simulink model "inverter_s1_kal"  (R2023b)
(part 2 of 3)

  N-Channel IGBT5 : ee_lib/Semiconductors & Converters/N-Channel IGBT  Commented=on  model_type=ee.enum.igbt.parameterization.equation  Ices=2 mA  Vces=600 V  Vth=6 V  Vce_sat=2.6 V  Ice_sat=400 A  Vge_sat=10 V  Tmeas=25 degC  Vge_vec=[-1, 0, 2, 3, 5, 6, 7, 8, 10, 12, 15, 18, 20] V  Vce_vec=[0, .25, .5, .75, 1, 1.26, 1.51, 1.76, 2.01, 2.26, 2.51, 2.76, 3.01, 3.27, 3.52, 3.77, 4.02, 4.27, 4.52, 4.77] V  T_vec=[25, 125] degC  Ic_mat=[0, 0, 0, 0, 0, 0, 0, 0, 0, 0, 0, 0, 0, 0, 0, 0, 0, 0, 0, 0; 0, 0, 0, 0, 0, 0, 0, 0, 0, 0, 0, 0, 0, 0, 0, 0, 0, 0, 0, 0; 0, 0, 0, 0, 0, 0, 0, 0, 0, 0, 0, 0, 0, 0, 0, 0, 0, 0, 0, 0; 0, 0, 0, 0, 0, 0, 0, 0, 0, 0, 0, 0, 0, 0, 0, 0, 0, 0, 0, 0; 0, 0, 0, 0, 0, 0, 0, 0, 0, 0, 0, 0, 0, 0, 0, 0, 0, 0, 0, 0; 0, 0, 0, .81, 3.13, 4.97, 6.03, 6.53, 6.84, 7.01, 7.19, 7.32, 7.44, 7.55, 7.67, 7.78, 7.89, 8, 8.07, 8.07; 0, 0, 0, 1.07, 5.5, 12.93, 22.09, 29.14, 35.27, 38.97, 41.37, 43.08, 44.52, 45.45, 46.28, 46.85, 47.41, 47.76, 48.06, 48.36; 0, 0, 0, 1.1, 6.99, 16.51, 28.38, 41.53, 55.76, 69.08, 80.5, 89.56, 96.13, 101.45, 105.15, 107.99, 110.09, 111.87, 113.54, 114.95; 0, 0, 0, 1.36, 6.26, 17.43, 33.6, 50.43, 71.75, 93.61, 114.64, 134.42, 151.44, 164.25, 177.06, 189.88, 202.69, 215.51, 228.32, 241.14; 0, 0, 0, 1.42, 6.4, 18.7, 36.19, 55.23, 79.71, 106.22, 131.28, 156.62, 182.79, 208.97, 235.15, 261.32, 287.5, 313.67, 339.85, 366.02; 0, 0, 0, 1.45, 6.81, 20.01, 39.61, 60.63, 88.74, 117.7, 147.16, 191.87, 237.14, 282.42, 327.69, 372.96, 418.23, 463.5, 508.77, 554.04; 0, 0, 0, 1.49, 6.97, 20.55, 41.34, 64.15, 94.91, 126.1, 170.16, 233.77, 297.38, 360.98, 424.59, 488.19, 551.8, 615.4, 679.01, 742.62; 0, 0, 0, 1.5, 7.5, 20.96, 42.17, 66.19, 98.34, 131.14, 187.84, 263.46, 339.09, 414.72, 490.34, 565.97, 641.6, 717.22, 792.85, 868.48] A  Ic_mat_3D=zeros(13, 20, 2) A  C_param=ee.enum.igbt.capacitanceParam.fixedciss  C_GE=23.7 nF  C_GC=2.7 nF  C_CE=0 nF  C_ies=26.4 nF  C_res=2.7 nF  C_oes=0 nF  C_GE_vec=[25, 31, 26.5, 24.9, 25, 24.9, 24.6, 24.7, 24.8] nF  C_GC_vec=[55, 9, 5.5, 3.1, 2.5, 2.1, 1.9, 1.8, 1.7] nF  C_Vge_vec=0 V  C_CE_vec=[5, 11, 6.5, 4.9, 3.5, 2.7, 2.1, 1.7, 1.4] nF  C_ies_vec=[80, 40, 32, 28, 27.5, 27, 26.5, 26.5, 26.5] nF  C_res_vec=[55, 9, 5.5, 3.1, 2.5, 2.1, 1.9, 1.8, 1.7] nF  C_oes_vec=[60, 20, 12, 8, 6, 4.8, 4, 3.5, 3.1] nF  C_Vce_vec=[0, 1, 2, 5, 10, 15, 20, 25, 30] V  charge_linearity_param=ee.enum.igbt.cgcLinearity.constant  C_OX=20 nF  V_C_OX=-5 V  TF=0 us  TT=0 us  ec=1  VAF=200 V  RC=0.001 Ohm  RE=0.001 Ohm  RG=0.001 Ohm  BF=50  T_param=ee.enum.igbt.temperatureParameterization.none  Ices_T2=100 mA  EG=1.11 eV  Vce_sat_T2=3 V  Tmeas2=125 degC  XTI=3  BEX=-1.5  RG_alpha=0 1/K  Tdevice=Tj_operating_K K  Tdevice_3D=25 degC  has_thermal_port=1  ig_specify=off  ig_priority=None  ig=0 A  ig_nominal_specify=off  ig_nominal_unit=A  ig_nominal_value=1  ic_specify=off  ic_priority=None  ic=0 A  ic_nominal_specify=off  ic_nominal_unit=A  ic_nominal_value=1  vge_specify=off  vge_priority=None  vge=0 V  vge_nominal_specify=off  vge_nominal_unit=V  vge_nominal_value=1  vce_specify=off  vce_priority=None  vce=0 V  vce_nominal_specify=off  vce_nominal_unit=V  vce_nominal_value=1  v_Cge_specify=off  v_Cge_priority=High  v_Cge=0 V  v_Cge_nominal_specify=off  v_Cge_nominal_unit=V  v_Cge_nominal_value=1  v_Cce_specify=off  v_Cce_priority=High  v_Cce=0 V  v_Cce_nominal_specify=off  v_Cce_nominal_unit=V  v_Cce_nominal_value=1  thermal_network_parameterization=ee.enum.thermalNetworkTopology.junctionCase  Rth=[0, 10] K/W  Rth_Cauer=[1, 3, 10] K/W  Rth_Foster=[4, 6] K/W  thermal_mass_parameterization=ee.enum.thermalNetwork.timeconstant  thermal_mass=[0, 1] J/K  thermal_mass_Cauer=[.1, .3, 1] J/K  thermal_mass_Foster=[1.5, 3] J/K  thermal_time_constant=[0, 10] s  thermal_time_constant_Cauer=[1, 3, 10] s  thermal_time_constant_Foster=[6, 18] s  thermal_mass_initial_temperatures=[25, 25] degC  thermal_mass_initial_temperatures_Cauer=[25, 25, 25] degC  Tvec_initial_Foster=[25, 25, 25, 25] degC  Ic_vec1=S12_Ic_cond A  Vce_vec1=[0, 1.1, 1.3, 1.45, 1.75, 2.25, 2.7] V  Rmiller=S12_Rmiller Ohm  Goff=S12_Goff 1/Ohm  t_on=S12_tondly s  t_rise=S12_risetime s  t_off=S12_toffdly s  t_fall=S12_falltime s  v_meas=S12_Voff_ref V  vStartTurnOn_specify=off  vStartTurnOn_priority=None  vStartTurnOn=1 V  tStartTurnOn_specify=off  tStartTurnOn_priority=None  tStartTurnOn=0 s  vStartTurnOff_specify=off  vStartTurnOff_priority=None  vStartTurnOff=0.5 V  tStartTurnOff_specify=off  tStartTurnOff_priority=None  tStartTurnOff=0 s  Tj_vec1=S12_Tj_cond K  Vce_mat1=S12_Vce_cond V  Tj_vec_loss=S12_Tj_loss K  Ic_vec_loss=S12_Ic_loss A  E_turn_on_mat1=S12_Eon J  E_turn_off_mat1=S12_Eoff J  iStartTurnOff_specify=off  iStartTurnOff_priority=None  iStartTurnOff=0 A  Tdevice_specify=off  Tdevice_priority=None
      settings: InternalSimscapePortConfiguration="{\"Bottom\":[],\"Left\":[{\"id\":\"G\",\"label\":\"\",\"type\":\"foundation.electrical.electrical\"},{\"id\":\"H\",\"label\":\"\",\"type\":\"foundation.thermal.thermal\"}],\"Right\":[{\"id\":\"C\",\"label\":\"\",\"type\":\"foundation.electrical.electrical\"},{\"id\":\"E\",\"label\":\"\",\"type\":\"foundation.electrical.electrical\"}],\"Top\":[]}"
  N-Channel IGBT6 : ee_lib/Semiconductors & Converters/N-Channel IGBT  Commented=on  model_type=ee.enum.igbt.parameterization.equation  Ices=2 mA  Vces=600 V  Vth=6 V  Vce_sat=2.6 V  Ice_sat=400 A  Vge_sat=10 V  Tmeas=25 degC  Vge_vec=[-1, 0, 2, 3, 5, 6, 7, 8, 10, 12, 15, 18, 20] V  Vce_vec=[0, .25, .5, .75, 1, 1.26, 1.51, 1.76, 2.01, 2.26, 2.51, 2.76, 3.01, 3.27, 3.52, 3.77, 4.02, 4.27, 4.52, 4.77] V  T_vec=[25, 125] degC  Ic_mat=[0, 0, 0, 0, 0, 0, 0, 0, 0, 0, 0, 0, 0, 0, 0, 0, 0, 0, 0, 0; 0, 0, 0, 0, 0, 0, 0, 0, 0, 0, 0, 0, 0, 0, 0, 0, 0, 0, 0, 0; 0, 0, 0, 0, 0, 0, 0, 0, 0, 0, 0, 0, 0, 0, 0, 0, 0, 0, 0, 0; 0, 0, 0, 0, 0, 0, 0, 0, 0, 0, 0, 0, 0, 0, 0, 0, 0, 0, 0, 0; 0, 0, 0, 0, 0, 0, 0, 0, 0, 0, 0, 0, 0, 0, 0, 0, 0, 0, 0, 0; 0, 0, 0, .81, 3.13, 4.97, 6.03, 6.53, 6.84, 7.01, 7.19, 7.32, 7.44, 7.55, 7.67, 7.78, 7.89, 8, 8.07, 8.07; 0, 0, 0, 1.07, 5.5, 12.93, 22.09, 29.14, 35.27, 38.97, 41.37, 43.08, 44.52, 45.45, 46.28, 46.85, 47.41, 47.76, 48.06, 48.36; 0, 0, 0, 1.1, 6.99, 16.51, 28.38, 41.53, 55.76, 69.08, 80.5, 89.56, 96.13, 101.45, 105.15, 107.99, 110.09, 111.87, 113.54, 114.95; 0, 0, 0, 1.36, 6.26, 17.43, 33.6, 50.43, 71.75, 93.61, 114.64, 134.42, 151.44, 164.25, 177.06, 189.88, 202.69, 215.51, 228.32, 241.14; 0, 0, 0, 1.42, 6.4, 18.7, 36.19, 55.23, 79.71, 106.22, 131.28, 156.62, 182.79, 208.97, 235.15, 261.32, 287.5, 313.67, 339.85, 366.02; 0, 0, 0, 1.45, 6.81, 20.01, 39.61, 60.63, 88.74, 117.7, 147.16, 191.87, 237.14, 282.42, 327.69, 372.96, 418.23, 463.5, 508.77, 554.04; 0, 0, 0, 1.49, 6.97, 20.55, 41.34, 64.15, 94.91, 126.1, 170.16, 233.77, 297.38, 360.98, 424.59, 488.19, 551.8, 615.4, 679.01, 742.62; 0, 0, 0, 1.5, 7.5, 20.96, 42.17, 66.19, 98.34, 131.14, 187.84, 263.46, 339.09, 414.72, 490.34, 565.97, 641.6, 717.22, 792.85, 868.48] A  Ic_mat_3D=zeros(13, 20, 2) A  C_param=ee.enum.igbt.capacitanceParam.fixedciss  C_GE=23.7 nF  C_GC=2.7 nF  C_CE=0 nF  C_ies=26.4 nF  C_res=2.7 nF  C_oes=0 nF  C_GE_vec=[25, 31, 26.5, 24.9, 25, 24.9, 24.6, 24.7, 24.8] nF  C_GC_vec=[55, 9, 5.5, 3.1, 2.5, 2.1, 1.9, 1.8, 1.7] nF  C_Vge_vec=0 V  C_CE_vec=[5, 11, 6.5, 4.9, 3.5, 2.7, 2.1, 1.7, 1.4] nF  C_ies_vec=[80, 40, 32, 28, 27.5, 27, 26.5, 26.5, 26.5] nF  C_res_vec=[55, 9, 5.5, 3.1, 2.5, 2.1, 1.9, 1.8, 1.7] nF  C_oes_vec=[60, 20, 12, 8, 6, 4.8, 4, 3.5, 3.1] nF  C_Vce_vec=[0, 1, 2, 5, 10, 15, 20, 25, 30] V  charge_linearity_param=ee.enum.igbt.cgcLinearity.constant  C_OX=20 nF  V_C_OX=-5 V  TF=0 us  TT=0 us  ec=1  VAF=200 V  RC=0.001 Ohm  RE=0.001 Ohm  RG=0.001 Ohm  BF=50  T_param=ee.enum.igbt.temperatureParameterization.none  Ices_T2=100 mA  EG=1.11 eV  Vce_sat_T2=3 V  Tmeas2=125 degC  XTI=3  BEX=-1.5  RG_alpha=0 1/K  Tdevice=Tj_operating_K K  Tdevice_3D=25 degC  has_thermal_port=1  ig_specify=off  ig_priority=None  ig=0 A  ig_nominal_specify=off  ig_nominal_unit=A  ig_nominal_value=1  ic_specify=off  ic_priority=None  ic=0 A  ic_nominal_specify=off  ic_nominal_unit=A  ic_nominal_value=1  vge_specify=off  vge_priority=None  vge=0 V  vge_nominal_specify=off  vge_nominal_unit=V  vge_nominal_value=1  vce_specify=off  vce_priority=None  vce=0 V  vce_nominal_specify=off  vce_nominal_unit=V  vce_nominal_value=1  v_Cge_specify=off  v_Cge_priority=High  v_Cge=0 V  v_Cge_nominal_specify=off  v_Cge_nominal_unit=V  v_Cge_nominal_value=1  v_Cce_specify=off  v_Cce_priority=High  v_Cce=0 V  v_Cce_nominal_specify=off  v_Cce_nominal_unit=V  v_Cce_nominal_value=1  thermal_network_parameterization=ee.enum.thermalNetworkTopology.junctionCase  Rth=[0, 10] K/W  Rth_Cauer=[1, 3, 10] K/W  Rth_Foster=[4, 6] K/W  thermal_mass_parameterization=ee.enum.thermalNetwork.timeconstant  thermal_mass=[0, 1] J/K  thermal_mass_Cauer=[.1, .3, 1] J/K  thermal_mass_Foster=[1.5, 3] J/K  thermal_time_constant=[0, 10] s  thermal_time_constant_Cauer=[1, 3, 10] s  thermal_time_constant_Foster=[6, 18] s  thermal_mass_initial_temperatures=[25, 25] degC  thermal_mass_initial_temperatures_Cauer=[25, 25, 25] degC  Tvec_initial_Foster=[25, 25, 25, 25] degC  Ic_vec1=S34_Ic_cond A  Vce_vec1=[0, 1.1, 1.3, 1.45, 1.75, 2.25, 2.7] V  Rmiller=S34_Rmiller Ohm  Goff=S34_Goff 1/Ohm  t_on=S34_tondly s  t_rise=S34_risetime s  t_off=S34_toffdly s  t_fall=S34_falltime s  v_meas=S34_Voff_ref V  vStartTurnOn_specify=off  vStartTurnOn_priority=None  vStartTurnOn=1 V  tStartTurnOn_specify=off  tStartTurnOn_priority=None  tStartTurnOn=0 s  vStartTurnOff_specify=off  vStartTurnOff_priority=None  vStartTurnOff=0.5 V  tStartTurnOff_specify=off  tStartTurnOff_priority=None  tStartTurnOff=0 s  Tj_vec1=S34_Tj_cond K  Vce_mat1=S34_Vce_cond V  Tj_vec_loss=S34_Tj_loss K  Ic_vec_loss=S34_Ic_loss A  E_turn_on_mat1=S34_Eon J  E_turn_off_mat1=S34_Eoff J  iStartTurnOff_specify=off  iStartTurnOff_priority=None  iStartTurnOff=0 A  Tdevice_specify=off  Tdevice_priority=None
      settings: InternalSimscapePortConfiguration="{\"Bottom\":[],\"Left\":[{\"id\":\"G\",\"label\":\"\",\"type\":\"foundation.electrical.electrical\"},{\"id\":\"H\",\"label\":\"\",\"type\":\"foundation.thermal.thermal\"}],\"Right\":[{\"id\":\"C\",\"label\":\"\",\"type\":\"foundation.electrical.electrical\"},{\"id\":\"E\",\"label\":\"\",\"type\":\"foundation.electrical.electrical\"}],\"Top\":[]}"
  N-Channel IGBT7 : ee_lib/Semiconductors & Converters/N-Channel IGBT  Commented=on  model_type=ee.enum.igbt.parameterization.equation  Ices=2 mA  Vces=600 V  Vth=6 V  Vce_sat=2.6 V  Ice_sat=400 A  Vge_sat=10 V  Tmeas=25 degC  Vge_vec=[-1, 0, 2, 3, 5, 6, 7, 8, 10, 12, 15, 18, 20] V  Vce_vec=[0, .25, .5, .75, 1, 1.26, 1.51, 1.76, 2.01, 2.26, 2.51, 2.76, 3.01, 3.27, 3.52, 3.77, 4.02, 4.27, 4.52, 4.77] V  T_vec=[25, 125] degC  Ic_mat=[0, 0, 0, 0, 0, 0, 0, 0, 0, 0, 0, 0, 0, 0, 0, 0, 0, 0, 0, 0; 0, 0, 0, 0, 0, 0, 0, 0, 0, 0, 0, 0, 0, 0, 0, 0, 0, 0, 0, 0; 0, 0, 0, 0, 0, 0, 0, 0, 0, 0, 0, 0, 0, 0, 0, 0, 0, 0, 0, 0; 0, 0, 0, 0, 0, 0, 0, 0, 0, 0, 0, 0, 0, 0, 0, 0, 0, 0, 0, 0; 0, 0, 0, 0, 0, 0, 0, 0, 0, 0, 0, 0, 0, 0, 0, 0, 0, 0, 0, 0; 0, 0, 0, .81, 3.13, 4.97, 6.03, 6.53, 6.84, 7.01, 7.19, 7.32, 7.44, 7.55, 7.67, 7.78, 7.89, 8, 8.07, 8.07; 0, 0, 0, 1.07, 5.5, 12.93, 22.09, 29.14, 35.27, 38.97, 41.37, 43.08, 44.52, 45.45, 46.28, 46.85, 47.41, 47.76, 48.06, 48.36; 0, 0, 0, 1.1, 6.99, 16.51, 28.38, 41.53, 55.76, 69.08, 80.5, 89.56, 96.13, 101.45, 105.15, 107.99, 110.09, 111.87, 113.54, 114.95; 0, 0, 0, 1.36, 6.26, 17.43, 33.6, 50.43, 71.75, 93.61, 114.64, 134.42, 151.44, 164.25, 177.06, 189.88, 202.69, 215.51, 228.32, 241.14; 0, 0, 0, 1.42, 6.4, 18.7, 36.19, 55.23, 79.71, 106.22, 131.28, 156.62, 182.79, 208.97, 235.15, 261.32, 287.5, 313.67, 339.85, 366.02; 0, 0, 0, 1.45, 6.81, 20.01, 39.61, 60.63, 88.74, 117.7, 147.16, 191.87, 237.14, 282.42, 327.69, 372.96, 418.23, 463.5, 508.77, 554.04; 0, 0, 0, 1.49, 6.97, 20.55, 41.34, 64.15, 94.91, 126.1, 170.16, 233.77, 297.38, 360.98, 424.59, 488.19, 551.8, 615.4, 679.01, 742.62; 0, 0, 0, 1.5, 7.5, 20.96, 42.17, 66.19, 98.34, 131.14, 187.84, 263.46, 339.09, 414.72, 490.34, 565.97, 641.6, 717.22, 792.85, 868.48] A  Ic_mat_3D=zeros(13, 20, 2) A  C_param=ee.enum.igbt.capacitanceParam.fixedciss  C_GE=23.7 nF  C_GC=2.7 nF  C_CE=0 nF  C_ies=26.4 nF  C_res=2.7 nF  C_oes=0 nF  C_GE_vec=[25, 31, 26.5, 24.9, 25, 24.9, 24.6, 24.7, 24.8] nF  C_GC_vec=[55, 9, 5.5, 3.1, 2.5, 2.1, 1.9, 1.8, 1.7] nF  C_Vge_vec=0 V  C_CE_vec=[5, 11, 6.5, 4.9, 3.5, 2.7, 2.1, 1.7, 1.4] nF  C_ies_vec=[80, 40, 32, 28, 27.5, 27, 26.5, 26.5, 26.5] nF  C_res_vec=[55, 9, 5.5, 3.1, 2.5, 2.1, 1.9, 1.8, 1.7] nF  C_oes_vec=[60, 20, 12, 8, 6, 4.8, 4, 3.5, 3.1] nF  C_Vce_vec=[0, 1, 2, 5, 10, 15, 20, 25, 30] V  charge_linearity_param=ee.enum.igbt.cgcLinearity.constant  C_OX=20 nF  V_C_OX=-5 V  TF=0 us  TT=0 us  ec=1  VAF=200 V  RC=0.001 Ohm  RE=0.001 Ohm  RG=0.001 Ohm  BF=50  T_param=ee.enum.igbt.temperatureParameterization.none  Ices_T2=100 mA  EG=1.11 eV  Vce_sat_T2=3 V  Tmeas2=125 degC  XTI=3  BEX=-1.5  RG_alpha=0 1/K  Tdevice=Tj_operating_K K  Tdevice_3D=25 degC  has_thermal_port=1  ig_specify=off  ig_priority=None  ig=0 A  ig_nominal_specify=off  ig_nominal_unit=A  ig_nominal_value=1  ic_specify=off  ic_priority=None  ic=0 A  ic_nominal_specify=off  ic_nominal_unit=A  ic_nominal_value=1  vge_specify=off  vge_priority=None  vge=0 V  vge_nominal_specify=off  vge_nominal_unit=V  vge_nominal_value=1  vce_specify=off  vce_priority=None  vce=0 V  vce_nominal_specify=off  vce_nominal_unit=V  vce_nominal_value=1  v_Cge_specify=off  v_Cge_priority=High  v_Cge=0 V  v_Cge_nominal_specify=off  v_Cge_nominal_unit=V  v_Cge_nominal_value=1  v_Cce_specify=off  v_Cce_priority=High  v_Cce=0 V  v_Cce_nominal_specify=off  v_Cce_nominal_unit=V  v_Cce_nominal_value=1  thermal_network_parameterization=ee.enum.thermalNetworkTopology.junctionCase  Rth=[0, 10] K/W  Rth_Cauer=[1, 3, 10] K/W  Rth_Foster=[4, 6] K/W  thermal_mass_parameterization=ee.enum.thermalNetwork.timeconstant  thermal_mass=[0, 1] J/K  thermal_mass_Cauer=[.1, .3, 1] J/K  thermal_mass_Foster=[1.5, 3] J/K  thermal_time_constant=[0, 10] s  thermal_time_constant_Cauer=[1, 3, 10] s  thermal_time_constant_Foster=[6, 18] s  thermal_mass_initial_temperatures=[25, 25] degC  thermal_mass_initial_temperatures_Cauer=[25, 25, 25] degC  Tvec_initial_Foster=[25, 25, 25, 25] degC  Ic_vec1=S34_Ic_cond A  Vce_vec1=[0, 1.1, 1.3, 1.45, 1.75, 2.25, 2.7] V  Rmiller=S34_Rmiller Ohm  Goff=S34_Goff 1/Ohm  t_on=S34_tondly s  t_rise=S34_risetime s  t_off=S34_toffdly s  t_fall=S34_falltime s  v_meas=S34_Voff_ref V  vStartTurnOn_specify=off  vStartTurnOn_priority=None  vStartTurnOn=1 V  tStartTurnOn_specify=off  tStartTurnOn_priority=None  tStartTurnOn=0 s  vStartTurnOff_specify=off  vStartTurnOff_priority=None  vStartTurnOff=0.5 V  tStartTurnOff_specify=off  tStartTurnOff_priority=None  tStartTurnOff=0 s  Tj_vec1=S34_Tj_cond K  Vce_mat1=S34_Vce_cond V  Tj_vec_loss=S34_Tj_loss K  Ic_vec_loss=S34_Ic_loss A  E_turn_on_mat1=S34_Eon J  E_turn_off_mat1=S34_Eoff J  iStartTurnOff_specify=off  iStartTurnOff_priority=None  iStartTurnOff=0 A  Tdevice_specify=off  Tdevice_priority=None
      settings: InternalSimscapePortConfiguration="{\"Bottom\":[],\"Left\":[{\"id\":\"G\",\"label\":\"\",\"type\":\"foundation.electrical.electrical\"},{\"id\":\"H\",\"label\":\"\",\"type\":\"foundation.thermal.thermal\"}],\"Right\":[{\"id\":\"C\",\"label\":\"\",\"type\":\"foundation.electrical.electrical\"},{\"id\":\"E\",\"label\":\"\",\"type\":\"foundation.electrical.electrical\"}],\"Top\":[]}"
  PS-Simulink Converter : nesl_utility/PS-Simulink Converter  PhysicalDomain=network_engine_domain  SubClassName=ps_output  LeftPortType=input  RightPortType=output  PseudoPeriodic=off  Frequencies=[]  VectorFormat=1-D array  Unit=1  AffineConversion=off
  PS-Simulink Converter1 : nesl_utility/PS-Simulink Converter  PhysicalDomain=network_engine_domain  SubClassName=ps_output  LeftPortType=input  RightPortType=output  PseudoPeriodic=off  Frequencies=[]  VectorFormat=1-D array  Unit=1  AffineConversion=off
  PS-Simulink Converter2 : nesl_utility/PS-Simulink Converter  Commented=on  PhysicalDomain=network_engine_domain  SubClassName=ps_output  LeftPortType=input  RightPortType=output  PseudoPeriodic=off  Frequencies=[]  VectorFormat=1-D array  Unit=1  AffineConversion=off
  PS-Simulink Converter3 : nesl_utility/PS-Simulink Converter  PhysicalDomain=network_engine_domain  SubClassName=ps_output  LeftPortType=input  RightPortType=output  PseudoPeriodic=off  Frequencies=[]  VectorFormat=1-D array  Unit=1  AffineConversion=off
  PS-Simulink Converter4 : nesl_utility/PS-Simulink Converter  Commented=on  PhysicalDomain=network_engine_domain  SubClassName=ps_output  LeftPortType=input  RightPortType=output  PseudoPeriodic=off  Frequencies=[]  VectorFormat=1-D array  Unit=1  AffineConversion=off
  PS-Simulink Converter5 : nesl_utility/PS-Simulink Converter  Commented=on  PhysicalDomain=network_engine_domain  SubClassName=ps_output  LeftPortType=input  RightPortType=output  PseudoPeriodic=off  Frequencies=[]  VectorFormat=1-D array  Unit=1  AffineConversion=off
  Power Measurement : eePowerMeasurement/Power Measurement  LabelModeActiveChoice=Continuous  F=50  K=0:50  Ts=0
  Power Measurement1 : eePowerMeasurement/Power Measurement  Commented=on  LabelModeActiveChoice=Continuous  F=50  K=0:50  Ts=0
  Power1 : spsPowerLib/Power  Commented=on  Freq=50  Vinit=[0.001, 0]  Iinit=[0.001, 0]  Ts=0
  Power3 : spsPowerLib/Power  Freq=50  Vinit=[0.001, 0]  Iinit=[0.001, 0]  Ts=0
  RMS1 : spsRMSLib/RMS  TrueRMS=on  Freq=50  RMSInit=0  Ts=0
  RMS2 : spsRMSLib/RMS  Commented=on  TrueRMS=on  Freq=50  RMSInit=0  Ts=0
  Resistor : ee_lib/Passive/Resistor  R=Rdc Ohm  enable_R_tol=ee.enum.toleranceApplication.none  R_tol=5  tol_distribution=ee.enum.toleranceDistribution.uniform  nSigma=4  enable_operating_limits=ee.enum.enable.no  operating_limit_action=ee.enum.passive.reportOpLim.warn  power_rating=1 W  max_working_voltage=100 V  enable_faults=ee.enum.enable.no  fault_action=simscape.enum.assert.action.none  R_faulted=inf Ohm  fault_trigger=ee.enum.faults.faultTrigger.temporal  t_fault=1 s  max_permissible_current=1 A  t_fail_on_current=1 s  noise_mode=ee.enum.sources.noise.Disabled  Tdevice=25 degC  sample_time=1e-3 s  repeatability=ee.enum.ic.repeatability.notRepeatable  user_seed=0  auto_seed=4112460543  faulted_specify=off  faulted_priority=None  faulted=0  power_derating_T1=70 degC  power_derating_T2=155 degC  operating_temperature_range_vec=[-50, 150] degC  alpha=3.93e-3 1/K  Tmeas=25 degC  thermal_mass=100 J/K  temperature_specify=off  temperature_priority=High  temperature=298.15 K  temperature_nominal_specify=off  temperature_nominal_unit=K  temperature_nominal_value=1
  Resistor1 : ee_lib/Passive/Resistor  R=R_bleed_1 Ohm  enable_R_tol=ee.enum.toleranceApplication.none  R_tol=5  tol_distribution=ee.enum.toleranceDistribution.uniform  nSigma=4  enable_operating_limits=ee.enum.enable.no  operating_limit_action=ee.enum.passive.reportOpLim.warn  power_rating=1 W  max_working_voltage=100 V  enable_faults=ee.enum.enable.no  fault_action=simscape.enum.assert.action.none  R_faulted=inf Ohm  fault_trigger=ee.enum.faults.faultTrigger.temporal  t_fault=1 s  max_permissible_current=1 A  t_fail_on_current=1 s  noise_mode=ee.enum.sources.noise.Disabled  Tdevice=25 degC  sample_time=1e-3 s  repeatability=ee.enum.ic.repeatability.notRepeatable  user_seed=0  auto_seed=4144164703  faulted_specify=off  faulted_priority=None  faulted=0  power_derating_T1=70 degC  power_derating_T2=155 degC  operating_temperature_range_vec=[-50, 150] degC  alpha=3.93e-3 1/K  Tmeas=25 degC  thermal_mass=100 J/K  temperature_specify=off  temperature_priority=High  temperature=298.15 K  temperature_nominal_specify=off  temperature_nominal_unit=K  temperature_nominal_value=1
  Resistor2 : ee_lib/Passive/Resistor  R=R_bleed_2 Ohm  enable_R_tol=ee.enum.toleranceApplication.none  R_tol=5  tol_distribution=ee.enum.toleranceDistribution.uniform  nSigma=4  enable_operating_limits=ee.enum.enable.no  operating_limit_action=ee.enum.passive.reportOpLim.warn  power_rating=1 W  max_working_voltage=100 V  enable_faults=ee.enum.enable.no  fault_action=simscape.enum.assert.action.none  R_faulted=inf Ohm  fault_trigger=ee.enum.faults.faultTrigger.temporal  t_fault=1 s  max_permissible_current=1 A  t_fail_on_current=1 s  noise_mode=ee.enum.sources.noise.Disabled  Tdevice=25 degC  sample_time=1e-3 s  repeatability=ee.enum.ic.repeatability.notRepeatable  user_seed=0  auto_seed=676943032  faulted_specify=off  faulted_priority=None  faulted=0  power_derating_T1=70 degC  power_derating_T2=155 degC  operating_temperature_range_vec=[-50, 150] degC  alpha=3.93e-3 1/K  Tmeas=25 degC  thermal_mass=100 J/K  temperature_specify=off  temperature_priority=High  temperature=298.15 K  temperature_nominal_specify=off  temperature_nominal_unit=K  temperature_nominal_value=1
  Resistor3 : ee_lib/Passive/Resistor  Commented=on  R=Rdc Ohm  enable_R_tol=ee.enum.toleranceApplication.none  R_tol=5  tol_distribution=ee.enum.toleranceDistribution.uniform  nSigma=4  enable_operating_limits=ee.enum.enable.no  operating_limit_action=ee.enum.passive.reportOpLim.warn  power_rating=1 W  max_working_voltage=100 V  enable_faults=ee.enum.enable.no  fault_action=simscape.enum.assert.action.none  R_faulted=inf Ohm  fault_trigger=ee.enum.faults.faultTrigger.temporal  t_fault=1 s  max_permissible_current=1 A  t_fail_on_current=1 s  noise_mode=ee.enum.sources.noise.Disabled  Tdevice=25 degC  sample_time=1e-3 s  repeatability=ee.enum.ic.repeatability.notRepeatable  user_seed=0  auto_seed=2348838240  faulted_specify=off  faulted_priority=None  faulted=0  power_derating_T1=70 degC  power_derating_T2=155 degC  operating_temperature_range_vec=[-50, 150] degC  alpha=3.93e-3 1/K  Tmeas=25 degC  thermal_mass=100 J/K  temperature_specify=off  temperature_priority=High  temperature=298.15 K  temperature_nominal_specify=off  temperature_nominal_unit=K  temperature_nominal_value=1
  Resistor4 : ee_lib/Passive/Resistor  Commented=on  R=R_bleed_1 Ohm  enable_R_tol=ee.enum.toleranceApplication.none  R_tol=5  tol_distribution=ee.enum.toleranceDistribution.uniform  nSigma=4  enable_operating_limits=ee.enum.enable.no  operating_limit_action=ee.enum.passive.reportOpLim.warn  power_rating=1 W  max_working_voltage=100 V  enable_faults=ee.enum.enable.no  fault_action=simscape.enum.assert.action.none  R_faulted=inf Ohm  fault_trigger=ee.enum.faults.faultTrigger.temporal  t_fault=1 s  max_permissible_current=1 A  t_fail_on_current=1 s  noise_mode=ee.enum.sources.noise.Disabled  Tdevice=25 degC  sample_time=1e-3 s  repeatability=ee.enum.ic.repeatability.notRepeatable  user_seed=0  auto_seed=4112460543  faulted_specify=off  faulted_priority=None  faulted=0  power_derating_T1=70 degC  power_derating_T2=155 degC  operating_temperature_range_vec=[-50, 150] degC  alpha=3.93e-3 1/K  Tmeas=25 degC  thermal_mass=100 J/K  temperature_specify=off  temperature_priority=High  temperature=298.15 K  temperature_nominal_specify=off  temperature_nominal_unit=K  temperature_nominal_value=1
  Resistor5 : ee_lib/Passive/Resistor  Commented=on  R=R_bleed_2 Ohm  enable_R_tol=ee.enum.toleranceApplication.none  R_tol=5  tol_distribution=ee.enum.toleranceDistribution.uniform  nSigma=4  enable_operating_limits=ee.enum.enable.no  operating_limit_action=ee.enum.passive.reportOpLim.warn  power_rating=1 W  max_working_voltage=100 V  enable_faults=ee.enum.enable.no  fault_action=simscape.enum.assert.action.none  R_faulted=inf Ohm  fault_trigger=ee.enum.faults.faultTrigger.temporal  t_fault=1 s  max_permissible_current=1 A  t_fail_on_current=1 s  noise_mode=ee.enum.sources.noise.Disabled  Tdevice=25 degC  sample_time=1e-3 s  repeatability=ee.enum.ic.repeatability.notRepeatable  user_seed=0  auto_seed=4144164703  faulted_specify=off  faulted_priority=None  faulted=0  power_derating_T1=70 degC  power_derating_T2=155 degC  operating_temperature_range_vec=[-50, 150] degC  alpha=3.93e-3 1/K  Tmeas=25 degC  thermal_mass=100 J/K  temperature_specify=off  temperature_priority=High  temperature=298.15 K  temperature_nominal_specify=off  temperature_nominal_unit=K  temperature_nominal_value=1
  S2 Goto g12 : Goto  Commented=on  GotoTag=g12  TagVisibility=global
  S2 Goto g22 : Goto  Commented=on  GotoTag=g22  TagVisibility=global
  S2 Goto g32 : Goto  Commented=on  GotoTag=g32  TagVisibility=global
  S2 Goto g42 : Goto  Commented=on  GotoTag=g42  TagVisibility=global
  S2 K1 : Gain  Commented=on  Gain=K12
  S2 K3 : Gain  Commented=on  Gain=0
  S2 PWM susturma : Subsystem  Commented=on
  S2 Sine Wave : Sin  Commented=on  Amplitude=pwm_ref_amp  Frequency=2*pi*f_grid  Phase=phase_deg2*pi/180  SampleTime=pwm_ref_Ts
  S2 Sum : Sum  Commented=on  Inputs=|++
  S2 sin2 : Product  Commented=on
  S2 sin3 : Product  Commented=on
  Scope{1,3..4,6,8,16..17} (7 alike) : Scope
  Scope{2,5,7,10..15,18..20} (12 alike) : Scope  Commented=on
  Sine Wave1 : Sin  Amplitude=pwm_ref_amp  Frequency=2*pi*f_grid  Phase=phase_deg1*pi/180  SampleTime=pwm_ref_Ts
  Sine Wave2 : Sin  Commented=on  Amplitude=pwm_ref_amp  Frequency=2*pi*f_grid  Phase=phase_deg2*pi/180  SampleTime=pwm_ref_Ts
  Solver Configuration1 : nesl_utility/Solver Configuration  PhysicalDomain=network_engine_domain  SubClassName=solver  LeftPortType=input  RightPortType=generic  Tones=[]  Harmonics=[]  SimulateNoise=off  Profile=off  UseLocalSampling=off  EnableSwitchedLinearOptims=on  FrequencyDomain=off  UseCCode=off  RelTol=0.001  AbsTol=1e-06  MinStep=1e-09  ToWorkspace=off  RevertToSquareIcSolve=off  NumHomotopyIterations=100  PhasorMode=off  PhasorModeNumHarmonics=1  ConsistencySolver=NEWTON_FTOL  IndexReductionMethod=DerivativeReplacement  DoDC=off  ResidualTolerance=simscape_residual_tolerance  ConsistencyTolSource=GLOBAL  ConsistencyAbsTol=0.001  ConsistencyRelTol=0.001  ConsistencyTolFactor=0.001  UseLocalSolver=off  LocalSolverChoice=NE_TRAPEZOIDAL_ADVANCER  ResolveIndetEquations=on  FunctionEvalNumThread=1  LocalSolverSampleTime=1e-7  DoFixedCost=off  MaxNonlinIter=10  MaxModeIter=2  ComputeImpulses=off  ImpulseIterations=1  LinearAlgebra=auto  LinearAlgebraNumThread=0  EquationFormulation=NE_TIME_EF  DelaysMemoryBudget=1024  AutomaticFiltering=on  FilteringTimeConstant=0.001  PartitionStorageMethod=AS_NEEDED  PartitionMemoryBudget=1024  PartitionMethod=FAST  MultibodyUseLocalSolver=off  MultibodyLocalSolverChoice=ODE1  MultibodyLocalSolverSampleTime=0.001
  Solver Configuration2 : nesl_utility/Solver Configuration  Commented=on  PhysicalDomain=network_engine_domain  SubClassName=solver  LeftPortType=input  RightPortType=generic  Tones=[]  Harmonics=[]  SimulateNoise=off  Profile=off  UseLocalSampling=off  EnableSwitchedLinearOptims=on  FrequencyDomain=off  UseCCode=off  RelTol=0.001  AbsTol=1e-06  MinStep=1e-09  ToWorkspace=off  RevertToSquareIcSolve=off  NumHomotopyIterations=100  PhasorMode=off  PhasorModeNumHarmonics=1  ConsistencySolver=NEWTON_FTOL  IndexReductionMethod=DerivativeReplacement  DoDC=off  ResidualTolerance=simscape_residual_tolerance  ConsistencyTolSource=GLOBAL  ConsistencyAbsTol=0.001  ConsistencyRelTol=0.001  ConsistencyTolFactor=0.001  UseLocalSolver=off  LocalSolverChoice=NE_TRAPEZOIDAL_ADVANCER  ResolveIndetEquations=on  FunctionEvalNumThread=1  LocalSolverSampleTime=1e-7  DoFixedCost=off  MaxNonlinIter=10  MaxModeIter=2  ComputeImpulses=off  ImpulseIterations=1  LinearAlgebra=auto  LinearAlgebraNumThread=0  EquationFormulation=NE_TIME_EF  DelaysMemoryBudget=1024  AutomaticFiltering=on  FilteringTimeConstant=0.001  PartitionStorageMethod=AS_NEEDED  PartitionMemoryBudget=1024  PartitionMethod=FAST  MultibodyUseLocalSolver=off  MultibodyLocalSolverChoice=ODE1  MultibodyLocalSolverSampleTime=0.001
  Sqrt : Sqrt
  Sqrt1 : Sqrt  Commented=on
  Sqrt2 : Sqrt
  Sqrt3 : Sqrt  Commented=on
  Subsystem : Subsystem
  Subsystem1 : Subsystem  Commented=on
  Sum of Elements : Sum  Inputs=+
  Sum of Elements1 : Sum  Inputs=+
  Sum of Elements2 : Sum  Commented=on  Inputs=+
  Sum of Elements3 : Sum  Commented=on  Inputs=+
  THD : spsTHDLib/THD  Freq=50  Ts=0
  THD1 : spsTHDLib/THD  Commented=on  Freq=50  Ts=0
  THD2 : spsTHDLib/THD  Freq=50  Ts=0
  THD3 : spsTHDLib/THD  Commented=on  Freq=50  Ts=0
  Temperature Source{,1..9} (10 alike) : fl_lib/Thermal/Thermal Sources/Temperature Source  temperature=25 degC
  Temperature Source{10..19} (10 alike) : fl_lib/Thermal/Thermal Sources/Temperature Source  Commented=on  temperature=25 degC
  Vdc : Display
  Vdc1 : Display  Commented=on
  Verim : Display
  Verim1 : Display  Commented=on
  Voltage Sensor : fl_lib/Electrical/Electrical Sensors/Voltage Sensor
      settings: LogSimulationData=on
  Voltage Sensor1 : fl_lib/Electrical/Electrical Sensors/Voltage Sensor  Commented=on
      settings: LogSimulationData=on
  Voltage Source : ee_lib/Sources/Voltage Source  dc_voltage=Vdc1 V  ac_voltage=0 V  ac_shift=0 rad  ac_frequency=50 Hz  noise_mode=ee.enum.sources.noise.Disabled  PSD=0 V^2/Hz  sample_time=1e-3 s  repeatability=ee.enum.sources.repeatability.NotRepeatable  user_seed=0  auto_seed=4168664255  i_specify=off  i_priority=None  i=0 A  i_nominal_specify=off  i_nominal_unit=A  i_nominal_value=1  v_specify=off  v_priority=None  v=0 V  v_nominal_specify=off  v_nominal_unit=V  v_nominal_value=1
  Voltage Source1 : ee_lib/Sources/Voltage Source  Commented=on  dc_voltage=Vdc2 V  ac_voltage=0 V  ac_shift=0 rad  ac_frequency=50 Hz  noise_mode=ee.enum.sources.noise.Disabled  PSD=0 V^2/Hz  sample_time=1e-3 s  repeatability=ee.enum.sources.repeatability.NotRepeatable  user_seed=0  auto_seed=676943032  i_specify=off  i_priority=None  i=0 A  i_nominal_specify=off  i_nominal_unit=A  i_nominal_value=1  v_specify=off  v_priority=None  v=0 V  v_nominal_specify=off  v_nominal_unit=V  v_nominal_value=1
  cosfi{,2..4} (4 alike) : Display
  cosfi{1,5..7} (4 alike) : Display  Commented=on
  powergui : spspowerguiLib/powergui  Priority=1  SimulationMode=Continuous  SampleTime=50e-6  frequency=50  Iterations=50  frequencyindice=60  Pbase=100e6  ErrMax=1e-4  UnitsV=kV  UnitsW=MW  buscounter=0  FunctionMessages=off  echomessages=off  EnableUseOfTLC=off  CurrentSourceSwitches=on  DisableSnubberDevices=off  DisableRonSwitches=off  DisableVfSwitches=off  DisplayEquations=off  AutomaticDiscreteSolvers=off  SolverType=Tustin/Backward Euler (TBE)  Interpol=off  ExternalGateDelay=off  methode=off  Ts=100  x0status=blocks  SPID=on  SwTol=0  HookPort=off  NonlinearTolerance=1e-4  nMaxIteration=100  ContinueOnMaxIteration=off  RestoreLinks=warning  ResistiveCurrentMeasurement=off  Frange=[0:2:500]  Ylog=off  Xlog=on  ShowGrid=off  save=off  variable=ZData  structure=0  ZoomFFT=off  StartTime=0.0  cycles=1  DisplayStyle=1  fundamental=50  FreqAxis=off  MaxFrequency=1000  frequencyindicesteady=1  RmsSteady=1  display=off
  tag scope: G11=global, G21=global, G31=global, G41=global, g11=global, g21=global, g31=global, g41=global, i_dc1=global, v_dc1=global
  wires:
  PS-Simulink Converter/1 -> [i_dc1]
  PS-Simulink Converter1/1 -> [v_dc1]
  From3/1 -> Bus Creator1/2
  Bus Creator1/1 -> Scope5/1
  From11/1 -> Bus Creator3/2, Bus Creator1/3
  Bus Creator2/1 -> Scope1/1
  Bus Creator3/1 -> Scope2/1
  [i_dc1] -> Bus Creator4/2
  Bus Creator4/1 -> Scope3/1
  [i_ac1] -> Power Measurement/2, THD/1, RMS1/1
  THD/1 -> AC Akım THD/1  "THD_s1"
  Mean1/1 -> Divide3/2, DC Güç/1
  AC instantaneous power/1 -> Mean1/1
  RMS1/1 -> AC Akım RMS/1  "Iac_s1"
  [v_ac1] -> THD2/1, Power Measurement/1
  [v_dc1] -> Bus Creator4/1
  [v_dc1] -> Mean2/1, AC instantaneous power/1
  [i_dc1] -> Mean3/1, AC instantaneous power/2
  Divide3/1 -> Verim/1  "eff_s1"
  Gain1/1 -> Bus Creator2/2
  [i_ac1] -> Gain1/1
  [v_ac1] -> Bus Creator2/1
  Mean2/1 -> Vdc/1  "Vdc_s1"
  Mean3/1 -> Idc/1  "Idc_s1"
  Sqrt/1 -> Divide1/2
  Add/1 -> Sqrt/1
  AC instantaneous power1/1 -> Add/1
  AC instantaneous power2/1 -> Add/2
  Divide1/1 -> cosfi/1  "cos_s1"
  Gate Drive7/1(G1) -> [G11]
  From1/1 -> Bus Creator3/1, Bus Creator1/1
  From12/1 -> Bus Creator1/4
  Gate Drive8/1(G4) -> [G41]
  Gate Drive5/1(G3) -> [G31]
  Gate Drive6/1(G2) -> [G21]
  [i_ac1] -> Scope4/1
  [v_inv1] -> Scope6/1
  PS-Simulink Converter3/1 -> Scope8/1
  Subsystem/2(Out2) -> [g21]
  Subsystem/4(Out4) -> [g41]
  Subsystem/1(Out1) -> [g11]
  Subsystem/3(Out3) -> [g31]
  Sine Wave1/1 -> K11/1
  K11/1 -> Subsystem/1(In1)
  K12/1 -> Subsystem1/1(In1)
  Sine Wave2/1 -> K12/1
  Subsystem1/3(Out3) -> Goto10/1
  Subsystem1/1(Out1) -> Goto4/1
  Subsystem1/4(Out4) -> Goto11/1
  Subsystem1/2(Out2) -> Goto8/1
  Subsystem/5(Out5) -> Bus Creator9/1
  Bus Creator9/1 -> Scope15/1
  Subsystem/6(Out6) -> Bus Creator9/2
  [v_ac1] -> Power3/1
  [i_ac1] -> Power3/2
  Divide5/1 -> cosfi4/1  "cos_s1"
  AC instantaneous power7/1 -> Add2/2
  AC instantaneous power6/1 -> Add2/1
  Add2/1 -> Sqrt2/1
  Sqrt2/1 -> Divide5/2
  Power3/2 -> AC instantaneous power6/1, AC instantaneous power6/2, cosfi3/1  "Q_s1"
  Power3/1 -> Scope17/1, AC instantaneous power7/1, AC instantaneous power7/2, Divide5/1, cosfi2/1  "P_s1"
  Mean9/1 -> AC Aktif Güç/1, Divide1/1, AC instantaneous power2/2, AC instantaneous power2/1, Divide3/1  "P_s1"
  Mean10/1 -> AC instantaneous power1/2, AC instantaneous power1/1, AC Reaktif Güç/1  "Q_s1"
  Power Measurement/1 -> Bus Creator10/2, Sum of Elements/1  "P_s1"
  Sum of Elements/1 -> Bus Creator10/1, Mean9/1
  Sum of Elements1/1 -> Mean10/1
  Power Measurement/2 -> Sum of Elements1/1  "Q_s1"
  Bus Creator10/1 -> Scope16/1
  THD2/1 -> AC Gerilim THD2/1  "THD_s1"
  From28/1 -> Power Measurement1/2, THD1/1, RMS2/1
  From32/1 -> Mean6/1, AC instantaneous power3/1
  AC instantaneous power9/1 -> Add3/2
  Mean4/1 -> Divide4/2, DC Güç1/1
  From17/1 -> Bus Creator8/2, Bus Creator5/3
  Power Measurement1/2 -> Sum of Elements3/1  "Q_s1"
  Add3/1 -> Sqrt3/1
  Add1/1 -> Sqrt1/1
  THD3/1 -> AC Gerilim THD1/1  "THD_s1"
  Power Measurement1/1 -> Bus Creator6/2, Sum of Elements2/1  "P_s1"
  Power1/2 -> AC instantaneous power8/1, AC instantaneous power8/2, cosfi6/1  "Q_s1"
  Sum of Elements2/1 -> Bus Creator6/1, Mean8/1
  Sum of Elements3/1 -> Mean5/1
  Mean8/1 -> AC Aktif Güç1/1, Divide2/1, AC instantaneous power5/2, AC instantaneous power5/1, Divide4/1  "P_s1"
  Sqrt1/1 -> Divide2/2
  From20/1 -> Scope19/1
  AC instantaneous power8/1 -> Add3/1
  Sqrt3/1 -> Divide6/2
  Power1/1 -> Scope11/1, AC instantaneous power9/1, AC instantaneous power9/2, Divide6/1, cosfi5/1  "P_s1"
  From18/1 -> Bus Creator5/4
  From22/1 -> Power1/2
  From24/1 -> Power1/1
  From16/1 -> Mean7/1, AC instantaneous power3/2
  From15/1 -> Bus Creator8/1, Bus Creator5/1
  Bus Creator7/1 -> Scope7/1
  Bus Creator5/1 -> Scope18/1
  Bus Creator8/1 -> Scope12/1
  From23/1 -> Bus Creator5/2
  Gain2/1 -> Bus Creator7/2
  Bus Creator6/1 -> Scope10/1
  Gate Drive2/1(G2) -> G8/1
  PS-Simulink Converter5/1 -> Scope20/1
  Divide2/1 -> cosfi1/1  "cos_s1"
  Gate Drive4/1(G4) -> G6/1
  Divide6/1 -> cosfi7/1  "cos_s1"
  From19/1 -> Scope14/1
  Mean5/1 -> AC instantaneous power4/2, AC instantaneous power4/1, AC Reaktif Güç1/1  "Q_s1"
  Mean7/1 -> Idc1/1  "Idc_s1"
  AC instantaneous power5/1 -> Add1/2
  Mean6/1 -> Vdc1/1  "Vdc_s1"
  RMS2/1 -> AC Akım RMS1/1  "Iac_s1"
  Gate Drive3/1(G1) -> G5/1
  From31/1 -> THD3/1, Power Measurement1/1
  Bus Creator11/1 -> Scope13/1
  Divide4/1 -> Verim1/1  "eff_s1"
  PS-Simulink Converter4/1 -> Goto3/1
  From27/1 -> Bus Creator11/2
  From25/1 -> Bus Creator7/1
  From21/1 -> Gain2/1
  From26/1 -> Bus Creator11/1
  THD1/1 -> AC Akım THD1/1  "THD_s1"
  AC instantaneous power3/1 -> Mean4/1
  PS-Simulink Converter2/1 -> Goto2/1
  AC instantaneous power4/1 -> Add1/1
  Gate Drive1/1(G3) -> G7/1
  S2 Sine Wave/1 -> S2 K1/1, S2 sin2/1, S2 sin2/2, S2 sin3/2
  S2 sin2/1 -> S2 sin3/1
  S2 sin3/1 -> S2 K3/1
  S2 K1/1 -> S2 Sum/1
  S2 K3/1 -> S2 Sum/2
  S2 Sum/1 -> S2 PWM susturma/1(In1)
  S2 PWM susturma/1(Out1) -> S2 Goto g12/1
  S2 PWM susturma/2(Out2) -> S2 Goto g22/1
  S2 PWM susturma/3(Out3) -> S2 Goto g32/1
  S2 PWM susturma/4(Out4) -> S2 Goto g42/1
  connections:
  Resistor1/RConn1 -- Capacitor/RConn1 -- Resistor2/LConn1 -- Capacitor1/LConn1 -- N-Channel IGBT2/RConn1 -- Diode6/RConn1 -- AC Voltage Sensor2/LConn1 -- EMC Common Mode Choke S1/RConn2 -- EMC Core Loss R1_2/RConn1 -- Capacitor2/RConn1
  Capacitor2/LConn1 -- EMC Common Mode Choke S1/LConn2 -- EMC Core Loss R1_1/RConn1 -- L1 Core Loss Rp/RConn1 -- Inductor/RConn1
  Capacitor1/RConn1 -- Resistor2/RConn1 -- N-Channel IGBT1/RConn2 -- Diode2/LConn1 -- Gate Drive6/RConn2 -- Diode3/LConn1 -- Voltage Sensor/RConn2 -- Voltage Source/RConn1 -- Electrical Reference1/LConn1 -- Solver Configuration1/RConn1
  Diode5/RConn1 -- Current Sensor/RConn2 -- Voltage Sensor/LConn1 -- Resistor1/LConn1 -- Capacitor/LConn1 -- N-Channel IGBT/RConn1 -- Diode9/RConn1
  N-Channel IGBT3/RConn1 -- Diode7/RConn1 -- Diode3/RConn1 -- Current Sensor1/LConn1 -- Resistor/LConn1 -- Diode5/LConn1
  Diode6/LConn1 -- N-Channel IGBT2/RConn2 -- N-Channel IGBT3/RConn2 -- Diode7/LConn1 -- Gate Drive5/RConn1 -- Gate Drive8/RConn2
  PS-Simulink Converter/LConn1 -- Current Sensor/RConn1
  Voltage Sensor/RConn1 -- PS-Simulink Converter1/LConn1
  Resistor/RConn1 -- Diode9/LConn1 -- Gate Drive7/RConn2 -- N-Channel IGBT/RConn2 -- N-Channel IGBT1/RConn1 -- Diode2/RConn1
  N-Channel IGBT3/LConn1 -- Gate Drive5/RConn2
  N-Channel IGBT1/LConn1 -- Gate Drive6/RConn1
  N-Channel IGBT2/LConn1 -- Gate Drive8/RConn1
  N-Channel IGBT/LConn1 -- Gate Drive7/RConn1
  Temperature Source/LConn1 -- Diode5/LConn2
  Temperature Source1/LConn1 -- Diode9/LConn2
  Diode2/LConn2 -- Temperature Source2/LConn1
  N-Channel IGBT1/LConn2 -- Temperature Source3/LConn1
  N-Channel IGBT/LConn2 -- Temperature Source4/LConn1
  Diode3/LConn2 -- Temperature Source5/LConn1
  N-Channel IGBT2/LConn2 -- Temperature Source6/LConn1
  N-Channel IGBT3/LConn2 -- Temperature Source7/LConn1
  Temperature Source8/LConn1 -- Diode6/LConn2
  Temperature Source9/LConn1 -- Diode7/LConn2
  Inductor/LConn1 -- L1 Core Loss Rp/LConn1 -- Current Sensor1/RConn2 -- AC Voltage Sensor2/RConn1
  PS-Simulink Converter3/LConn1 -- Current Sensor1/RConn1
  Voltage Source/LConn1 -- DC Blocking Diode/LConn1
  DC Blocking Diode/RConn1 -- DC Source R/LConn1
  DC Source R/RConn1 -- Current Sensor/LConn1
  CL1/RConn1 -- Grid1/LConn1
  Grid1/RConn1 -- AC Current Sensor1/RConn1 -- AC Voltage Sensor1/LConn1
  CL1/LConn1 -- EMC Common Mode Choke S3/LConn1 -- EMC Core Loss R2_1/LConn1 -- AC Voltage Sensor1/RConn1
  EMC Common Mode Choke S1/RConn1 -- Capacitor6/RConn1 -- EMC Common Mode Choke S3/RConn2 -- EMC Core Loss R2_2/RConn1 -- EMC Core Loss R1_2/LConn1
  EMC Common Mode Choke S1/LConn1 -- EMC Core Loss R1_1/LConn1 -- EMC Common Mode Choke S3/LConn2 -- EMC Core Loss R2_1/RConn1 -- Capacitor6/LConn1
  EMC Common Mode Choke S3/RConn1 -- EMC Core Loss R2_2/LConn1 -- AC Current Sensor1/RConn2
  Capacitor3/LConn1 -- Resistor4/LConn1 -- Diode8/RConn1 -- N-Channel IGBT4/RConn1 -- Diode12/RConn1 -- Current Sensor2/RConn2 -- Voltage Sensor1/LConn1
  N-Channel IGBT4/RConn2 -- Resistor3/RConn1 -- N-Channel IGBT5/RConn1 -- Diode1/RConn1 -- Diode12/LConn1 -- Gate Drive3/RConn2
  EMC Core Loss R2_4/RConn1 -- Capacitor7/RConn1 -- EMC Common Mode Choke S2/RConn1 -- EMC Core Loss R1_4/LConn1 -- EMC Common Mode Choke S4/RConn2
  Capacitor3/RConn1 -- EMC Common Mode Choke S2/RConn2 -- EMC Core Loss R1_4/RConn1 -- Capacitor5/RConn1 -- AC Voltage Sensor4/LConn1 -- Resistor5/LConn1 -- Capacitor4/LConn1 -- N-Channel IGBT6/RConn1 -- Diode10/RConn1 -- Resistor4/RConn1
  Gate Drive2/RConn2 -- Capacitor4/RConn1 -- Resistor5/RConn1 -- Voltage Sensor1/RConn2 -- Voltage Source1/RConn1 -- Electrical Reference2/LConn1 -- Solver Configuration2/RConn1 -- Diode4/LConn1 -- N-Channel IGBT5/RConn2 -- Diode1/LConn1
  AC Voltage Sensor4/RConn1 -- Inductor1/LConn1 -- L1 Core Loss Rp1/LConn1 -- Current Sensor3/RConn2
  AC Current Sensor2/RConn2 -- EMC Common Mode Choke S4/RConn1 -- EMC Core Loss R2_4/LConn1
  Diode11/LConn1 -- Diode10/LConn1 -- N-Channel IGBT6/RConn2 -- Gate Drive4/RConn2 -- Gate Drive1/RConn1 -- N-Channel IGBT7/RConn2
  Resistor3/LConn1 -- N-Channel IGBT7/RConn1 -- Diode11/RConn1 -- Diode4/RConn1 -- Diode8/LConn1 -- Current Sensor3/LConn1
  Inductor1/RConn1 -- Capacitor5/LConn1 -- EMC Common Mode Choke S2/LConn2 -- EMC Core Loss R1_3/RConn1 -- L1 Core Loss Rp1/RConn1
  EMC Core Loss R2_3/LConn1 -- CL2/LConn1 -- AC Voltage Sensor3/RConn1 -- EMC Common Mode Choke S4/LConn1
  EMC Core Loss R2_3/RConn1 -- EMC Common Mode Choke S2/LConn1 -- EMC Core Loss R1_3/LConn1 -- Capacitor7/LConn1 -- EMC Common Mode Choke S4/LConn2
  AC Voltage Sensor3/LConn1 -- AC Current Sensor2/RConn1 -- Grid2/RConn1
  Diode4/LConn2 -- Temperature Source15/LConn1
  CL2/RConn1 -- Grid2/LConn1
  Diode1/LConn2 -- Temperature Source12/LConn1
  N-Channel IGBT7/LConn2 -- Temperature Source17/LConn1
  N-Channel IGBT5/LConn2 -- Temperature Source13/LConn1
  Temperature Source10/LConn1 -- Diode8/LConn2
  DC Source R1/RConn1 -- Current Sensor2/LConn1
  N-Channel IGBT7/LConn1 -- Gate Drive1/RConn2
  PS-Simulink Converter5/LConn1 -- Current Sensor3/RConn1
  Voltage Source1/LConn1 -- DC Blocking Diode1/LConn1
  N-Channel IGBT6/LConn2 -- Temperature Source16/LConn1
  Temperature Source18/LConn1 -- Diode10/LConn2
  Temperature Source11/LConn1 -- Diode12/LConn2
  Temperature Source19/LConn1 -- Diode11/LConn2
  N-Channel IGBT4/LConn2 -- Temperature Source14/LConn1
  Voltage Sensor1/RConn1 -- PS-Simulink Converter4/LConn1
  N-Channel IGBT6/LConn1 -- Gate Drive4/RConn1
  DC Blocking Diode1/RConn1 -- DC Source R1/LConn1
  N-Channel IGBT4/LConn1 -- Gate Drive3/RConn1
  N-Channel IGBT5/LConn1 -- Gate Drive2/RConn1
  PS-Simulink Converter2/LConn1 -- Current Sensor2/RConn1
